simulink model "Formation_control"  (R2025a)
settings: Solver=VariableStepAuto  StartTime=0.0  StopTime=10.0  RelTol=1e-3
InitFcn:
  | %% Simulation parameters and waypoint trajectory
  | % Initial drone positions.
  | init_0=[0;0;0];
  | d_s=4;
  | init_1=init_0+d_s*[-1.1;0.1;0];
  | init_2=init_0+d_s*[0.3;-1.5;0];
  | init_3=init_0+d_s*[1.6;0.4;0];
  | init_4=init_0+d_s*[0.2;1.8;0];
  | 
  | Threshold = 1000*ones(45,1);
  | for i=1:9:37
  |     Threshold(i:i+2)=10;
  | end
  | gain_2=1;
  | 
  | % Desired formation offsets.
  | init_f_0=[0;0;0];
  | d_f=1.5;
  | init_f_1=init_0+d_f*[1;0;0];
  | init_f_2=init_0+d_f*[0;1;0];
  | init_f_3=init_0+d_f*[-1;0;0];
  | init_f_4=init_0+d_f*[0;-1;0];
  | % Quadrotor mass and inertia.
  | mass = 1.2;
  | Ib   = diag([1.2416 1.2416 2*1.2416]);
  | 
  | % Time grid and waypoint trajectory.
  | Ts        = 0.001;
  | ttot      = 20;
  | tdead     = 10;
  | totalTime = ttot + tdead;
  | Nsamples  = 3000;
  | t_sample  = linspace(0, totalTime, Nsamples);
  | t=t_sample;
  | waypoints = [ ...
  |      0    0   -2        0;
  |    3  4  -5    0;
  |    2  1  -3     0;
  |      0    0   0 0];
  | 
  | M    = size(waypoints,1);
  | t_wp = linspace(0, ttot, M);
  | 
  | p_d      = zeros(4, Nsamples);
  | dot_p_d  = zeros(4, Nsamples);
  | ddot_p_d = zeros(4, Nsamples);
  | 
  | idx_traj = t_sample <= ttot;
  | t_active = t_sample(idx_traj);
  | 
  | % Build position and yaw splines with zero endpoint velocities.
  | for dim = 1:4
  |     pp  = spline(t_wp, [0, waypoints(:,dim)&apos;, 0]);
  |     pp1 = fnder(pp,1);
  |     pp2 = fnder(pp,2);
  | 
  |     p_d(dim,    idx_traj) = ppval(pp,  t_active);
  |     dot_p_d(dim,idx_traj) = ppval(pp1, t_active);
  |     ddot_p_d(dim,idx_traj)= ppval(pp2, t_active);
  | end
  | ... (+19 lines)
undefined symbols (not defined in the file): A_diacenza, K
libraries: robotcorelib x5, uavutilslib x1
(part 2 of 2)

== system Formation_control/Subsystem1/Subsystem_5/Quadrotor dynamics ==
  uT : Inport
  tau_b : Inport  Port=2
  Integrator : Integrator  InitialCondition=init_4
  Integrator1 : Integrator  InitialCondition=lin_vel_0
  Integrator2 : Integrator  InitialCondition=[1 0 0; 0 1 0;0 0 1]
  Integrator3 : Integrator  InitialCondition=w_bb_0
  MATLAB Function1 : MATLAB Function  TreatAsAtomicUnit=on
  UAV dynamics : MATLAB Function  TreatAsAtomicUnit=on
  Position : Outport
  Linear_velocity : Outport  Port=2
  Rb : Outport  Port=3
  dot_Rb : Outport  Port=4
  omega_bb : Outport  Port=5
  dot_omega_bb : Outport  Port=6
  lin_acc : Outport  Port=7
  wires:
  Integrator2/1 -> MATLAB Function1/1(Rb_temp)
  MATLAB Function1/1(Rb) -> UAV dynamics/3(Rb), Rb/1
  UAV dynamics/2(dot_Rb) -> dot_Rb/1, Integrator2/1
  Integrator3/1 -> omega_bb/1, UAV dynamics/4(omega_bb)
  Integrator1/1 -> Integrator/1, Linear_velocity/1
  uT/1 -> UAV dynamics/1(uT)
  UAV dynamics/1(lin_acc) -> Integrator1/1, lin_acc/1
  UAV dynamics/3(ang_acc) -> Integrator3/1, dot_omega_bb/1
  Integrator/1 -> Position/1
  tau_b/1 -> UAV dynamics/2(tau_b)

== matlab function Formation_control/Subsystem1/Subsystem_2/Inner-loop control/Inner-loop control ==
  data: Rb_des output size=[3,3]; omega_bb_des output size=3; tau output size=3; zb_des input size=3; Rb input size=[3,3]; dot_Rb_des input size=[3,3]; omega_bb input size=3; dot_omega_bb_des input size=3; xb_des input size=3; Ib parameter size=[3,3]; err_R output size=3; err_W output size=3
function [Rb_des,omega_bb_des,tau,err_R,err_W] = fcn(zb_des,Rb,dot_Rb_des,omega_bb,dot_omega_bb_des,xb_des,Ib)
% Geometric attitude control from rotation and angular-velocity errors.


k_rx = 50;
k_ry = 50;
k_rz = 50;

k_wx = 50;
k_wy = 50;
k_wz = 50;

K_r = diag([k_rx, k_ry, k_rz]);
K_w = diag([k_wx, k_wy, k_wz]);


% Construct the desired rotation matrix from the requested body axes.
yb_des = (skew(zb_des)*xb_des)/norm(skew(zb_des)*xb_des);

Rb_des = [skew(yb_des)*zb_des, yb_des, zb_des];

omega_bb_des = wedge(Rb_des&apos;*dot_Rb_des);

err_R = 0.5*wedge(Rb_des&apos;*Rb - Rb&apos;*Rb_des);

err_W = omega_bb - Rb&apos;*Rb_des*omega_bb_des;

% Combine attitude feedback with rigid-body compensation.
tau = -K_r*err_R - K_w*err_W + skew(omega_bb)*Ib*omega_bb - Ib*(skew(omega_bb)*Rb&apos;*Rb_des*omega_bb_des-Rb&apos;*Rb_des*dot_omega_bb_des); 

end

function S = skew(v)
% Matrix representation of the cross product.
if(numel(v)~= 1)
S= [0 -v(3) v(2); 
    v(3) 0 -v(1);
    -v(2) v(1) 0];
else
S= zeros(3);
end
end

function v = wedge(S)
% Extract the vector associated with a skew-symmetric matrix.
v1 = S(3,2);
v2 = S(1,3);
v3 = S(2,1);
v = [v1 v2 v3]&apos;;
end

== matlab function Formation_control/Subsystem1/Subsystem_2/Outer-loop control ==
  data: position input size=3; uT output size=1; linear_vel input size=3; Rb input size=[3,3]; zb_des output size=3; mass parameter size=1; position_des input size=3; vel_linear_des input size=3; acc_linear_des input size=3; err_p output size=3; dot_err_p output size=3
function [uT, zb_des, err_p, dot_err_p] = fcn(position, linear_vel, Rb, mass, ...
    position_des, vel_linear_des, acc_linear_des)
% Outer-loop position control: compute thrust and the desired body z-axis.


k_px = 10;
k_py = 10;
k_pz = 20;

k_vx = 10;
k_vy = 10;
k_vz = 20;

K_p = diag([k_px, k_py, k_pz]);
K_v = diag([k_vx, k_vy, k_vz]);


g = 9.81;

e_3 = [0 0 1]&apos;;

err_p = position - position_des;

dot_err_p = linear_vel - vel_linear_des;

% Normalize the commanded force to obtain the desired thrust direction.
zb_des = -(-K_p*err_p-K_v*dot_err_p-mass*g*e_3+mass*acc_linear_des)/norm(-K_p*err_p-K_v*dot_err_p-mass*g*e_3+mass*acc_linear_des);

uT = -(-K_p*err_p-K_v*dot_err_p-mass*g*e_3+mass*acc_linear_des)&apos;*Rb*e_3;

== matlab function Formation_control/Subsystem1/Subsystem_2/Quadrotor dynamics/MATLAB Function1 ==
  data: Rb_temp input; Rb output
function Rb = fcn(Rb_temp)
% Project the integrated matrix back onto SO(3) using SVD.
    [U,S,V] = svd(Rb_temp);
    sigma = det(U*V&apos;);
    S_ = diag([1 1 sigma]);

    Rb = U*S_*V&apos;;
end

== matlab function Formation_control/Subsystem1/Subsystem_2/Quadrotor dynamics/UAV dynamics ==
  data: uT input size=1; tau_b input size=3; lin_acc output size=3; Rb input size=[3,3]; omega_bb input size=3; dot_Rb output size=[3,3]; ang_acc output size=3; mass parameter size=1; Ib parameter size=[3,3]
function [lin_acc, dot_Rb, ang_acc] = fcn(uT,tau_b,Rb,omega_bb,mass, Ib)
% Quadrotor translational and rotational rigid-body dynamics.

lin_acc = 9.81*[0 0 1]&apos;-(uT/mass)*Rb*[0 0 1]&apos;;
dot_Rb = Rb*skew(omega_bb);
ang_acc = inv(Ib)*(-skew(omega_bb)*Ib*omega_bb + tau_b);

end

function S = skew(v)
% Matrix representation of the cross product.
if(numel(v)~= 1)
S= [0 -v(3) v(2); 
    v(3) 0 -v(1);
    -v(2) v(1) 0];
else
S= zeros(3);
end
end

== matlab function Formation_control/Subsystem1/Subsystem_3/Inner-loop control/Inner-loop control ==
  data: Rb_des output size=[3,3]; omega_bb_des output size=3; tau output size=3; zb_des input size=3; Rb input size=[3,3]; dot_Rb_des input size=[3,3]; omega_bb input size=3; dot_omega_bb_des input size=3; xb_des input size=3; Ib parameter size=[3,3]; err_R output size=3; err_W output size=3
function [Rb_des,omega_bb_des,tau,err_R,err_W] = fcn(zb_des,Rb,dot_Rb_des,omega_bb,dot_omega_bb_des,xb_des,Ib)
% Geometric attitude control from rotation and angular-velocity errors.


k_rx = 50;
k_ry = 50;
k_rz = 50;

k_wx = 50;
k_wy = 50;
k_wz = 50;

K_r = diag([k_rx, k_ry, k_rz]);
K_w = diag([k_wx, k_wy, k_wz]);


% Construct the desired rotation matrix from the requested body axes.
yb_des = (skew(zb_des)*xb_des)/norm(skew(zb_des)*xb_des);

Rb_des = [skew(yb_des)*zb_des, yb_des, zb_des];

omega_bb_des = wedge(Rb_des&apos;*dot_Rb_des);

err_R = 0.5*wedge(Rb_des&apos;*Rb - Rb&apos;*Rb_des);

err_W = omega_bb - Rb&apos;*Rb_des*omega_bb_des;

% Combine attitude feedback with rigid-body compensation.
tau = -K_r*err_R - K_w*err_W + skew(omega_bb)*Ib*omega_bb - Ib*(skew(omega_bb)*Rb&apos;*Rb_des*omega_bb_des-Rb&apos;*Rb_des*dot_omega_bb_des); 

end

function S = skew(v)
% Matrix representation of the cross product.
if(numel(v)~= 1)
S= [0 -v(3) v(2); 
    v(3) 0 -v(1);
    -v(2) v(1) 0];
else
S= zeros(3);
end
end

function v = wedge(S)
% Extract the vector associated with a skew-symmetric matrix.
v1 = S(3,2);
v2 = S(1,3);
v3 = S(2,1);
v = [v1 v2 v3]&apos;;
end

== matlab function Formation_control/Subsystem1/Subsystem_3/Outer-loop control ==
  data: position input size=3; uT output size=1; linear_vel input size=3; Rb input size=[3,3]; zb_des output size=3; mass parameter size=1; position_des input size=3; vel_linear_des input size=3; acc_linear_des input size=3; err_p output size=3; dot_err_p output size=3
function [uT, zb_des, err_p, dot_err_p] = fcn(position, linear_vel, Rb, mass, ...
    position_des, vel_linear_des, acc_linear_des)
% Outer-loop position control: compute thrust and the desired body z-axis.


k_px = 10;
k_py = 10;
k_pz = 20;

k_vx = 10;
k_vy = 10;
k_vz = 20;

K_p = diag([k_px, k_py, k_pz]);
K_v = diag([k_vx, k_vy, k_vz]);


g = 9.81;

e_3 = [0 0 1]&apos;;

err_p = position - position_des;

dot_err_p = linear_vel - vel_linear_des;

% Normalize the commanded force to obtain the desired thrust direction.
zb_des = -(-K_p*err_p-K_v*dot_err_p-mass*g*e_3+mass*acc_linear_des)/norm(-K_p*err_p-K_v*dot_err_p-mass*g*e_3+mass*acc_linear_des);

uT = -(-K_p*err_p-K_v*dot_err_p-mass*g*e_3+mass*acc_linear_des)&apos;*Rb*e_3;

== matlab function Formation_control/Subsystem1/Subsystem_3/Quadrotor dynamics/MATLAB Function1 ==
  data: Rb_temp input; Rb output
function Rb = fcn(Rb_temp)
% Project the integrated matrix back onto SO(3) using SVD.
    [U,S,V] = svd(Rb_temp);
    sigma = det(U*V&apos;);
    S_ = diag([1 1 sigma]);

    Rb = U*S_*V&apos;;
end

== matlab function Formation_control/Subsystem1/Subsystem_3/Quadrotor dynamics/UAV dynamics ==
  data: uT input size=1; tau_b input size=3; lin_acc output size=3; Rb input size=[3,3]; omega_bb input size=3; dot_Rb output size=[3,3]; ang_acc output size=3; mass parameter size=1; Ib parameter size=[3,3]
function [lin_acc, dot_Rb, ang_acc] = fcn(uT,tau_b,Rb,omega_bb,mass, Ib)
% Quadrotor translational and rotational rigid-body dynamics.

lin_acc = 9.81*[0 0 1]&apos;-(uT/mass)*Rb*[0 0 1]&apos;;
dot_Rb = Rb*skew(omega_bb);
ang_acc = inv(Ib)*(-skew(omega_bb)*Ib*omega_bb + tau_b);

end

function S = skew(v)
% Matrix representation of the cross product.
if(numel(v)~= 1)
S= [0 -v(3) v(2); 
    v(3) 0 -v(1);
    -v(2) v(1) 0];
else
S= zeros(3);
end
end

== matlab function Formation_control/Subsystem1/Subsystem_4/Inner-loop control/Inner-loop control ==
  data: Rb_des output size=[3,3]; omega_bb_des output size=3; tau output size=3; zb_des input size=3; Rb input size=[3,3]; dot_Rb_des input size=[3,3]; omega_bb input size=3; dot_omega_bb_des input size=3; xb_des input size=3; Ib parameter size=[3,3]; err_R output size=3; err_W output size=3
function [Rb_des,omega_bb_des,tau,err_R,err_W] = fcn(zb_des,Rb,dot_Rb_des,omega_bb,dot_omega_bb_des,xb_des,Ib)
% Geometric attitude control from rotation and angular-velocity errors.


k_rx = 50;
k_ry = 50;
k_rz = 50;

k_wx = 50;
k_wy = 50;
k_wz = 50;

K_r = diag([k_rx, k_ry, k_rz]);
K_w = diag([k_wx, k_wy, k_wz]);


% Construct the desired rotation matrix from the requested body axes.
yb_des = (skew(zb_des)*xb_des)/norm(skew(zb_des)*xb_des);

Rb_des = [skew(yb_des)*zb_des, yb_des, zb_des];

omega_bb_des = wedge(Rb_des&apos;*dot_Rb_des);

err_R = 0.5*wedge(Rb_des&apos;*Rb - Rb&apos;*Rb_des);

err_W = omega_bb - Rb&apos;*Rb_des*omega_bb_des;

% Combine attitude feedback with rigid-body compensation.
tau = -K_r*err_R - K_w*err_W + skew(omega_bb)*Ib*omega_bb - Ib*(skew(omega_bb)*Rb&apos;*Rb_des*omega_bb_des-Rb&apos;*Rb_des*dot_omega_bb_des); 

end

function S = skew(v)
% Matrix representation of the cross product.
if(numel(v)~= 1)
S= [0 -v(3) v(2); 
    v(3) 0 -v(1);
    -v(2) v(1) 0];
else
S= zeros(3);
end
end

function v = wedge(S)
% Extract the vector associated with a skew-symmetric matrix.
v1 = S(3,2);
v2 = S(1,3);
v3 = S(2,1);
v = [v1 v2 v3]&apos;;
end

== matlab function Formation_control/Subsystem1/Subsystem_4/Outer-loop control ==
  data: position input size=3; uT output size=1; linear_vel input size=3; Rb input size=[3,3]; zb_des output size=3; mass parameter size=1; position_des input size=3; vel_linear_des input size=3; acc_linear_des input size=3; err_p output size=3; dot_err_p output size=3
function [uT, zb_des, err_p, dot_err_p] = fcn(position, linear_vel, Rb, mass, ...
    position_des, vel_linear_des, acc_linear_des)
% Outer-loop position control: compute thrust and the desired body z-axis.


k_px = 10;
k_py = 10;
k_pz = 20;

k_vx = 10;
k_vy = 10;
k_vz = 20;

K_p = diag([k_px, k_py, k_pz]);
K_v = diag([k_vx, k_vy, k_vz]);


g = 9.81;

e_3 = [0 0 1]&apos;;

err_p = position - position_des;

dot_err_p = linear_vel - vel_linear_des;

% Normalize the commanded force to obtain the desired thrust direction.
zb_des = -(-K_p*err_p-K_v*dot_err_p-mass*g*e_3+mass*acc_linear_des)/norm(-K_p*err_p-K_v*dot_err_p-mass*g*e_3+mass*acc_linear_des);

uT = -(-K_p*err_p-K_v*dot_err_p-mass*g*e_3+mass*acc_linear_des)&apos;*Rb*e_3;

== matlab function Formation_control/Subsystem1/Subsystem_4/Quadrotor dynamics/MATLAB Function1 ==
  data: Rb_temp input; Rb output
function Rb = fcn(Rb_temp)
% Project the integrated matrix back onto SO(3) using SVD.
    [U,S,V] = svd(Rb_temp);
    sigma = det(U*V&apos;);
    S_ = diag([1 1 sigma]);

    Rb = U*S_*V&apos;;
end

== matlab function Formation_control/MATLAB Function ==
  data: M input; vec output; V input
function vec = concatena_colonne(M, V)
% Stack state columns for the network controller.
    if ~isequal(size(M), [3,5]) || ~isequal(size(V), [3,5])
        error(&apos;Le matrici devono essere entrambe di dimensione 3x5.&apos;);
    end

    C = zeros(3, 10);

    C(:, 1:2:end) = M;
    C(:, 2:2:end) = V;

    vec = C(:);
end

== matlab function Formation_control/Subsystem1/Subsystem_4/Quadrotor dynamics/UAV dynamics ==
  data: uT input size=1; tau_b input size=3; lin_acc output size=3; Rb input size=[3,3]; omega_bb input size=3; dot_Rb output size=[3,3]; ang_acc output size=3; mass parameter size=1; Ib parameter size=[3,3]
function [lin_acc, dot_Rb, ang_acc] = fcn(uT,tau_b,Rb,omega_bb,mass, Ib)
% Quadrotor translational and rotational rigid-body dynamics.

lin_acc = 9.81*[0 0 1]&apos;-(uT/mass)*Rb*[0 0 1]&apos;;
dot_Rb = Rb*skew(omega_bb);
ang_acc = inv(Ib)*(-skew(omega_bb)*Ib*omega_bb + tau_b);

end

function S = skew(v)
% Matrix representation of the cross product.
if(numel(v)~= 1)
S= [0 -v(3) v(2); 
    v(3) 0 -v(1);
    -v(2) v(1) 0];
else
S= zeros(3);
end
end

== matlab function Formation_control/Subsystem1/Subsystem_5/Inner-loop control/Inner-loop control ==
  data: Rb_des output size=[3,3]; omega_bb_des output size=3; tau output size=3; zb_des input size=3; Rb input size=[3,3]; dot_Rb_des input size=[3,3]; omega_bb input size=3; dot_omega_bb_des input size=3; xb_des input size=3; Ib parameter size=[3,3]; err_R output size=3; err_W output size=3
function [Rb_des,omega_bb_des,tau,err_R,err_W] = fcn(zb_des,Rb,dot_Rb_des,omega_bb,dot_omega_bb_des,xb_des,Ib)
% Geometric attitude control from rotation and angular-velocity errors.


k_rx = 50;
k_ry = 50;
k_rz = 50;

k_wx = 50;
k_wy = 50;
k_wz = 50;

K_r = diag([k_rx, k_ry, k_rz]);
K_w = diag([k_wx, k_wy, k_wz]);


% Construct the desired rotation matrix from the requested body axes.
yb_des = (skew(zb_des)*xb_des)/norm(skew(zb_des)*xb_des);

Rb_des = [skew(yb_des)*zb_des, yb_des, zb_des];

omega_bb_des = wedge(Rb_des&apos;*dot_Rb_des);

err_R = 0.5*wedge(Rb_des&apos;*Rb - Rb&apos;*Rb_des);

err_W = omega_bb - Rb&apos;*Rb_des*omega_bb_des;

% Combine attitude feedback with rigid-body compensation.
tau = -K_r*err_R - K_w*err_W + skew(omega_bb)*Ib*omega_bb - Ib*(skew(omega_bb)*Rb&apos;*Rb_des*omega_bb_des-Rb&apos;*Rb_des*dot_omega_bb_des); 

end

function S = skew(v)
% Matrix representation of the cross product.
if(numel(v)~= 1)
S= [0 -v(3) v(2); 
    v(3) 0 -v(1);
    -v(2) v(1) 0];
else
S= zeros(3);
end
end

function v = wedge(S)
% Extract the vector associated with a skew-symmetric matrix.
v1 = S(3,2);
v2 = S(1,3);
v3 = S(2,1);
v = [v1 v2 v3]&apos;;
end

== matlab function Formation_control/Subsystem1/Subsystem_5/Outer-loop control ==
  data: position input size=3; uT output size=1; linear_vel input size=3; Rb input size=[3,3]; zb_des output size=3; mass parameter size=1; position_des input size=3; vel_linear_des input size=3; acc_linear_des input size=3; err_p output size=3; dot_err_p output size=3
function [uT, zb_des, err_p, dot_err_p] = fcn(position, linear_vel, Rb, mass, ...
    position_des, vel_linear_des, acc_linear_des)
% Outer-loop position control: compute thrust and the desired body z-axis.


k_px = 10;
k_py = 10;
k_pz = 20;

k_vx = 10;
k_vy = 10;
k_vz = 20;

K_p = diag([k_px, k_py, k_pz]);
K_v = diag([k_vx, k_vy, k_vz]);


g = 9.81;

e_3 = [0 0 1]&apos;;

err_p = position - position_des;

dot_err_p = linear_vel - vel_linear_des;

% Normalize the commanded force to obtain the desired thrust direction.
zb_des = -(-K_p*err_p-K_v*dot_err_p-mass*g*e_3+mass*acc_linear_des)/norm(-K_p*err_p-K_v*dot_err_p-mass*g*e_3+mass*acc_linear_des);

uT = -(-K_p*err_p-K_v*dot_err_p-mass*g*e_3+mass*acc_linear_des)&apos;*Rb*e_3;

== matlab function Formation_control/Subsystem1/Subsystem_5/Quadrotor dynamics/MATLAB Function1 ==
  data: Rb_temp input; Rb output
function Rb = fcn(Rb_temp)
% Project the integrated matrix back onto SO(3) using SVD.
    [U,S,V] = svd(Rb_temp);
    sigma = det(U*V&apos;);
    S_ = diag([1 1 sigma]);

    Rb = U*S_*V&apos;;
end

== matlab function Formation_control/Subsystem1/Subsystem_5/Quadrotor dynamics/UAV dynamics ==
  data: uT input size=1; tau_b input size=3; lin_acc output size=3; Rb input size=[3,3]; omega_bb input size=3; dot_Rb output size=[3,3]; ang_acc output size=3; mass parameter size=1; Ib parameter size=[3,3]
function [lin_acc, dot_Rb, ang_acc] = fcn(uT,tau_b,Rb,omega_bb,mass, Ib)
% Quadrotor translational and rotational rigid-body dynamics.

lin_acc = 9.81*[0 0 1]&apos;-(uT/mass)*Rb*[0 0 1]&apos;;
dot_Rb = Rb*skew(omega_bb);
ang_acc = inv(Ib)*(-skew(omega_bb)*Ib*omega_bb + tau_b);

end

function S = skew(v)
% Matrix representation of the cross product.
if(numel(v)~= 1)
S= [0 -v(3) v(2); 
    v(3) 0 -v(1);
    -v(2) v(1) 0];
else
S= zeros(3);
end
end

== matlab function Formation_control/MATLAB Function1 ==
  data: x input; alpha input; v_out output; A input
function v_out = controllo_repulsivo(x, alpha, A)
% Repulsive velocity correction from neighboring drone positions.

    N = 5;
    dim = 3;
    
    v_out = zeros(N * dim, 1);
    
    % Read position entries from the stacked state blocks.
    pos = zeros(dim, N);
    for i = 1:N
        idx = (i - 1) * 9 + 1;
        pos(:, i) = x(idx : idx + 2);
    end
    
    for i = 2:N
        vi = zeros(dim, 1);
        pi = pos(:, i);
        for j = 2:N
            if A(i, j) == 1 && i ~= j
                pj = pos(:, j);
                delta = pi - pj;
                norm_delta = norm(delta);
                if norm_delta > 0
                    vi = vi + 25*alpha*delta * exp(-alpha*(norm_delta-2))-0.00054*norm_delta*delta;
                end
            end
        end
        v_out((i-1)*dim + 1 : i*dim) = vi;
    end
end

== matlab function Formation_control/MATLAB Function2 ==
  data: M input; vec output; V input; A input
function vec = concatena_colonne(M, V, A)
% Stack state columns for the network controller.
    C = zeros(3, 15);

    C(:, 1:3:end) = M;
    C(:, 2:3:end) = V;
    C(:, 3:3:end) = A;

    vec = C(:);
end

== matlab function Formation_control/Subsystem1/Subsystem_1/Inner-loop control/Inner-loop control ==
  data: Rb_des output size=[3,3]; omega_bb_des output size=3; tau output size=3; zb_des input size=3; Rb input size=[3,3]; dot_Rb_des input size=[3,3]; omega_bb input size=3; dot_omega_bb_des input size=3; xb_des input size=3; Ib parameter size=[3,3]; err_R output size=3; err_W output size=3
function [Rb_des,omega_bb_des,tau,err_R,err_W] = fcn(zb_des,Rb,dot_Rb_des,omega_bb,dot_omega_bb_des,xb_des,Ib)
% Geometric attitude control from rotation and angular-velocity errors.


k_rx = 50;
k_ry = 50;
k_rz = 50;

k_wx = 50;
k_wy = 50;
k_wz = 50;

K_r = diag([k_rx, k_ry, k_rz]);
K_w = diag([k_wx, k_wy, k_wz]);


% Construct the desired rotation matrix from the requested body axes.
yb_des = (skew(zb_des)*xb_des)/norm(skew(zb_des)*xb_des);

Rb_des = [skew(yb_des)*zb_des, yb_des, zb_des];

omega_bb_des = wedge(Rb_des&apos;*dot_Rb_des);

err_R = 0.5*wedge(Rb_des&apos;*Rb - Rb&apos;*Rb_des);

err_W = omega_bb - Rb&apos;*Rb_des*omega_bb_des;

% Combine attitude feedback with rigid-body compensation.
tau = -K_r*err_R - K_w*err_W + skew(omega_bb)*Ib*omega_bb - Ib*(skew(omega_bb)*Rb&apos;*Rb_des*omega_bb_des-Rb&apos;*Rb_des*dot_omega_bb_des); 

end

function S = skew(v)
% Matrix representation of the cross product.
if(numel(v)~= 1)
S= [0 -v(3) v(2); 
    v(3) 0 -v(1);
    -v(2) v(1) 0];
else
S= zeros(3);
end
end

function v = wedge(S)
% Extract the vector associated with a skew-symmetric matrix.
v1 = S(3,2);
v2 = S(1,3);
v3 = S(2,1);
v = [v1 v2 v3]&apos;;
end

== matlab function Formation_control/Subsystem1/Subsystem_1/Outer-loop control ==
  data: position input size=3; uT output size=1; linear_vel input size=3; Rb input size=[3,3]; zb_des output size=3; mass parameter size=1; position_des input size=3; vel_linear_des input size=3; acc_linear_des input size=3; err_p output size=3; dot_err_p output size=3
function [uT, zb_des, err_p, dot_err_p] = fcn(position, linear_vel, Rb, mass, ...
    position_des, vel_linear_des, acc_linear_des)
% Outer-loop position control: compute thrust and the desired body z-axis.


k_px = 10;
k_py = 10;
k_pz = 20;

k_vx = 10;
k_vy = 10;
k_vz = 20;

K_p = diag([k_px, k_py, k_pz]);
K_v = diag([k_vx, k_vy, k_vz]);


g = 9.81;

e_3 = [0 0 1]&apos;;

err_p = position - position_des;

dot_err_p = linear_vel - vel_linear_des;

% Normalize the commanded force to obtain the desired thrust direction.
zb_des = -(-K_p*err_p-K_v*dot_err_p-mass*g*e_3+mass*acc_linear_des)/norm(-K_p*err_p-K_v*dot_err_p-mass*g*e_3+mass*acc_linear_des);

uT = -(-K_p*err_p-K_v*dot_err_p-mass*g*e_3+mass*acc_linear_des)&apos;*Rb*e_3;

== matlab function Formation_control/Subsystem1/Subsystem_1/Quadrotor dynamics/MATLAB Function1 ==
  data: Rb_temp input; Rb output
function Rb = fcn(Rb_temp)
% Project the integrated matrix back onto SO(3) using SVD.
    [U,S,V] = svd(Rb_temp);
    sigma = det(U*V&apos;);
    S_ = diag([1 1 sigma]);

    Rb = U*S_*V&apos;;
end

== matlab function Formation_control/Subsystem1/Subsystem_1/Quadrotor dynamics/UAV dynamics ==
  data: uT input size=1; tau_b input size=3; lin_acc output size=3; Rb input size=[3,3]; omega_bb input size=3; dot_Rb output size=[3,3]; ang_acc output size=3; mass parameter size=1; Ib parameter size=[3,3]
function [lin_acc, dot_Rb, ang_acc] = fcn(uT,tau_b,Rb,omega_bb,mass, Ib)
% Quadrotor translational and rotational rigid-body dynamics.

lin_acc = 9.81*[0 0 1]&apos;-(uT/mass)*Rb*[0 0 1]&apos;;
dot_Rb = Rb*skew(omega_bb);
ang_acc = inv(Ib)*(-skew(omega_bb)*Ib*omega_bb + tau_b);

end

function S = skew(v)
% Matrix representation of the cross product.
if(numel(v)~= 1)
S= [0 -v(3) v(2); 
    v(3) 0 -v(1);
    -v(2) v(1) 0];
else
S= zeros(3);
end
end
